simulink model "apf_offline"  (R2022b)
settings: Solver=VariableStepAuto  StartTime=0.0  StopTime=40  RelTol=1e-3
values from neighbouring files (symbols this model uses):
  d0 = 2.5    [apf_offline_script.m]
  g = 9.81    [apf_offline_script.m]
  Ib = diag([0.0347563 0.0458929 0.0977])    [apf_offline_script.m]
  initori = [0 0 0]    [scenario_generator.m]
  initpos = q_0    [scenario_generator.m]
  initvel = [0 0 0]    [scenario_generator.m]
  k_att = 0.8    [apf_offline_script.m]
  k_rep = 0.03    [apf_offline_script.m]
  kp = diag([6 6 6])    [apf_offline_script.m]
  kr = diag([2 2.3 0.15])    [apf_offline_script.m]
  kv = diag([4.7 4.7 4.7])    [apf_offline_script.m]
  kw = diag([0.4 0.52 0.18])    [apf_offline_script.m]
  mass = 1.52    [apf_offline_script.m]
  q_goal = [10 10 -10]    [apf_offline_script.m]
  q_obs1 = obs_points_gen(obs_1)    [apf_offline_script.m]
  q_obs2 = obs_points_gen(obs_2)    [apf_offline_script.m]
  q_obstacles = [obs_points_gen(obs_1); obs_points_gen(obs_2)]    [apf_offline_script.m]
  Ts = 0.001    [apf_offline_script.m]
  uT_0 = 14.92    [apf_offline_script.m]
libraries: uavsimlib x3, eeGeneralControl x1, robotcorelib x1
settings Model: VariantFading=off  Creator=The MathWorks, Inc.  LastModifiedBy=stefa
settings DebuggingCC: UnconnectedInputMsg=warning  UnconnectedOutputMsg=warning  UnconnectedLineMsg=warning
settings ModelReferenceCC: EnableRefExpFcnMdlSchedulingChecks=on
settings RTWCC: DLArmComputeVersion=19.05

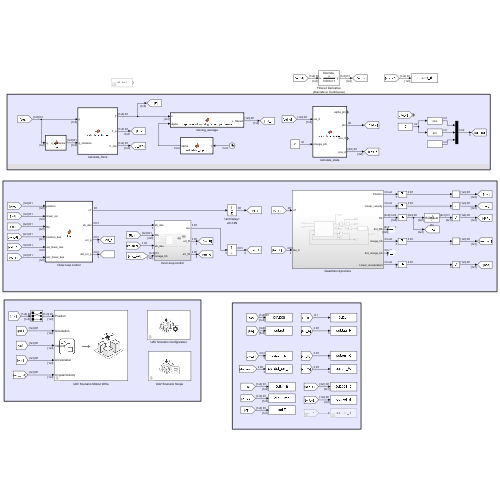
[thumbnail: Simulink's stored preview of the top-level diagram]
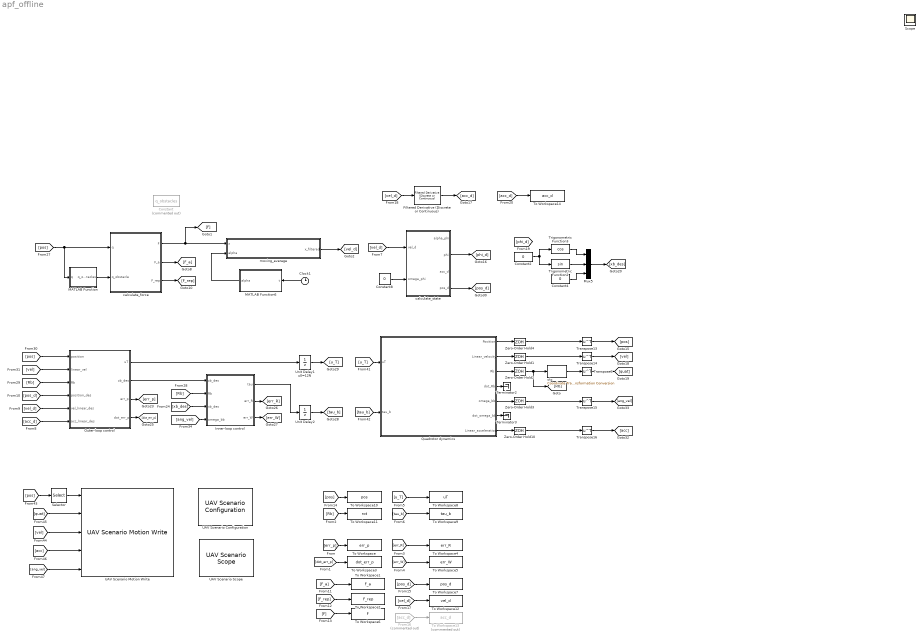
== system apf_offline ==
  Clock1 : Clock
  Constant : Constant  Commented=on  Value=q_obstacles
  Constant2 : Constant  Value=0
  Constant4 : Constant  Value=0
  Constant8 : Constant  Value=0
  Filtered Derivative (Discrete or Continuous) : eeGeneralControl/Filtered Derivative (Discrete or Continuous)  K=1  T=Ts  B=inf  A=-inf  minRatio=10  init_option=Specify as parameter  x0=[0 0 0]  Ts=-1
      settings: LibrarySourceBlock=|
      | ee_sl_lib/General Control/Filtered Derivative
      | (Discrete or Continuous)
  From16 : From  Commented=on  GotoTag=acc_d
  Inner-loop control : Subsystem
  MATLAB Function : MATLAB Function  TreatAsAtomicUnit=on
  MATLAB Function6 : MATLAB Function  TreatAsAtomicUnit=on
  Mux5 : Mux  Inputs=3
  Outer-loop control : MATLAB Function  TreatAsAtomicUnit=on
  Quadrotor dynamics : Subsystem
  Selector : Selector  InputPortWidth=3  IndexOptions=Index vector (dialog)  Indices=[2 1 3]  OutputSizes=1
  Terminator2 : Terminator
  Terminator3 : Terminator
  To Workspace : ToWorkspace  VariableName=err_p  SaveFormat=Timeseries  SampleTime=-1
  To Workspace1 : ToWorkspace  VariableName=F_a  SampleTime=-1
      settings: Save2DSignal=2-D array (concatenate along first dimension)
  To Workspace10 : ToWorkspace  VariableName=pos  SampleTime=-1
      settings: Save2DSignal=2-D array (concatenate along first dimension)
  To Workspace11 : ToWorkspace  VariableName=rot  SaveFormat=Timeseries  SampleTime=-1
  To Workspace12 : ToWorkspace  VariableName=vel_d  SampleTime=-1
      settings: Save2DSignal=2-D array (concatenate along first dimension)
  To Workspace13 : ToWorkspace  Commented=on  VariableName=acc_d  SampleTime=-1
  To Workspace14 : ToWorkspace  VariableName=acc_d  SampleTime=-1
      settings: Save2DSignal=2-D array (concatenate along first dimension)
  To Workspace2 : ToWorkspace  VariableName=F_rep  SampleTime=-1
      settings: Save2DSignal=2-D array (concatenate along first dimension)
  To Workspace3 : ToWorkspace  VariableName=dot_err_p  SaveFormat=Timeseries  SampleTime=-1
  To Workspace4 : ToWorkspace  VariableName=err_R  SaveFormat=Timeseries  SampleTime=-1
  To Workspace5 : ToWorkspace  VariableName=err_W  SaveFormat=Timeseries  SampleTime=-1
  To Workspace6 : ToWorkspace  VariableName=F  SampleTime=-1
      settings: Save2DSignal=2-D array (concatenate along first dimension)
  To Workspace7 : ToWorkspace  VariableName=pos_d  SampleTime=-1
  To Workspace8 : ToWorkspace  VariableName=uT  SaveFormat=Timeseries  SampleTime=-1
  To Workspace9 : ToWorkspace  VariableName=tau_b  SaveFormat=Timeseries  SampleTime=-1
  Transpose{6,13..16} (5 alike) : Math  Operator=transpose
  Trigonometric Function2 : Trigonometry
  Trigonometric Function3 : Trigonometry  Operator=cos
  UAV Scenario Configuration : uavsimlib/UAV Scenario Configuration  Priority=-1  UAVScenarioObject=scene  SampleTime=Ts  UpdateParam=true  SensorMotionBusName='SensorMotionBus'  PlatformMotionBusName='PlatformMotionBus'  ScenarioMotionBusName='ScenarioMotionBus'  ScenarioMotionSignalName='ScenarioMotions'
  UAV Scenario Motion Write : uavsimlib/UAV Scenario Motion Write  Priority=0  PlatName='platformUAV'  ReferenceFrame=NED
  UAV Scenario Scope : uavsimlib/UAV Scenario Scope  Priority=1  SensorNameTable={}  SampleTime=0.1
  Unit Delay1 u0=12N : UnitDelay  InitialCondition=uT_0  SampleTime=Ts
  Unit Delay2 : UnitDelay  InitialCondition=[0 0 0]  SampleTime=Ts
  Zero-Order Hold{1..4,10} (5 alike) : ZeroOrderHold  SampleTime=Ts
  calculate_force : MATLAB Function  TreatAsAtomicUnit=on
  calculate_state : MATLAB Function  TreatAsAtomicUnit=on
  ctc : robotcorelib/Coordinate Transformation Conversion  InputRepresentation=Rotation Matrix  InputEulerSequence=ZYX  ShowTrVecInputPort=on  OutputRepresentation=Quaternion  OutputEulerSequence=ZYX  ShowTrVecOutputPort=on  SimulateUsing=Interpreted execution
  moving_average : MATLAB Function  TreatAsAtomicUnit=on
  Scope : Scope
  wires:
  Trigonometric Function3/1 -> Mux5/1
  Constant4/1 -> Mux5/3
  Constant2/1 -> Trigonometric Function2/1, Trigonometric Function3/1
  Trigonometric Function2/1 -> Mux5/2
  Constant8/1 -> calculate_state/2(omega_phi)
  calculate_state/2(phi) -> [phi_d]
  MATLAB Function/1(q_obstacles) -> calculate_force/2(q_obstacle)
  calculate_force/1(F) -> [F], moving_average/1(x)
  Quadrotor dynamics/1(Position) -> Zero-Order Hold4/1
  Outer-loop control/2(zb_des) -> Inner-loop control/1(zb_des)
  Zero-Order Hold4/1 -> Transpose13/1
  Quadrotor dynamics/6(dot_omega_bb) -> Terminator3/1
  Quadrotor dynamics/5(omega_bb) -> Zero-Order Hold3/1
  [xb_des] -> Inner-loop control/3(xb_des)
  [vel_d] -> Outer-loop control/5(vel_linear_des)
  Quadrotor dynamics/4(dot_Rb) -> Terminator2/1
  Zero-Order Hold2/1 -> [Rb], ctc/1
  [acc_d] -> Outer-loop control/6(acc_linear_des)
  Inner-loop control/2(err_R) -> [err_R]
  Zero-Order Hold1/1 -> Transpose14/1
  Inner-loop control/3(err_W) -> [err_W]
  Inner-loop control/1(tau) -> Unit Delay2/1
  Unit Delay1 u0=12N/1 -> [u_T]
  Quadrotor dynamics/2(Linear_velocity) -> Zero-Order Hold1/1
  Unit Delay2/1 -> [tau_b]
  Outer-loop control/3(err_p) -> [err_p]
  Outer-loop control/1(uT) -> Unit Delay1 u0=12N/1
  [pos_d] -> Outer-loop control/4(position_des)
  Outer-loop control/4(dot_err_p) -> [dot_err_p]
  Quadrotor dynamics/3(Rb) -> Zero-Order Hold2/1
  ctc/1 -> Transpose6/1
  [pos] -> Selector/1
  [quat] -> UAV Scenario Motion Write/2
  [vel] -> UAV Scenario Motion Write/3
  Transpose6/1 -> [quat]
  [Rb] -> Inner-loop control/2(Rb)
  [Rb] -> Outer-loop control/3(Rb)
  [pos] -> Outer-loop control/1(position)
  [vel] -> Outer-loop control/2(linear_vel)
  [pos] -> MATLAB Function/1(q), calculate_force/1(q)
  calculate_state/4(pos_d) -> [pos_d]
  [vel_d] -> calculate_state/1(vel_d)
  calculate_force/3(F_rep) -> [F_rep]
  calculate_force/2(F_a) -> [F_a]
  [ang_vel] -> Inner-loop control/4(omega_bb)
  Mux5/1 -> [xb_des]
  [u_T] -> Quadrotor dynamics/1(uT)
  [tau_b] -> Quadrotor dynamics/2(tau_b)
  Transpose13/1 -> [pos]
  Transpose14/1 -> [vel]
  Transpose16/1 -> [acc]
  Zero-Order Hold10/1 -> Transpose16/1
  Quadrotor dynamics/7(Linear_acceleration) -> Zero-Order Hold10/1
  [acc] -> UAV Scenario Motion Write/4
  Zero-Order Hold3/1 -> Transpose15/1
  Transpose15/1 -> [ang_vel]
  [ang_vel] -> UAV Scenario Motion Write/5
  Clock1/1 -> MATLAB Function6/1(t)
  MATLAB Function6/1(alpha) -> moving_average/2(alpha)
  Selector/1 -> UAV Scenario Motion Write/1
  [tau_b] -> To Workspace9/1
  [err_p] -> To Workspace/1
  [pos] -> To Workspace10/1
  [dot_err_p] -> To Workspace3/1
  [u_T] -> To Workspace8/1
  [err_W] -> To Workspace5/1
  [err_R] -> To Workspace4/1
  [Rb] -> To Workspace11/1
  [F_rep] -> To Workspace2/1
  [F_a] -> To Workspace1/1
  [F] -> To Workspace6/1
  [pos_d] -> To Workspace7/1
  From16/1 -> To Workspace13/1
  [vel_d] -> To Workspace12/1
  moving_average/1(x_filtered) -> [vel_d]
  Filtered Derivative (Discrete or Continuous)/1 -> [acc_d]
  [vel_d] -> Filtered Derivative (Discrete or Continuous)/1
  [acc_d] -> To Workspace14/1

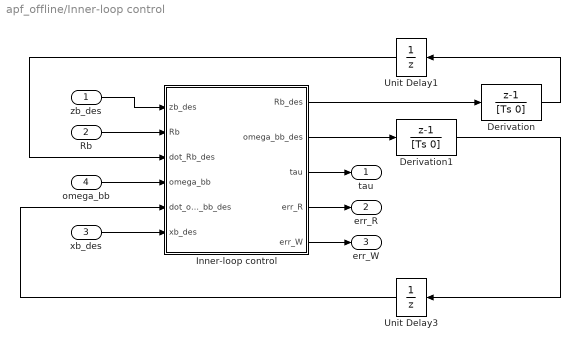
== system apf_offline/Inner-loop control ==
  zb_des : Inport
  Rb : Inport  Port=2
  xb_des : Inport  Port=3
  omega_bb : Inport  Port=4
  Derivation : DiscreteTransferFcn  Numerator=[1 -1]  Denominator=[Ts 0]  InitialStates=[1 0 0;0 1 0;0 0 1]  SampleTime=Ts
  Derivation1 : DiscreteTransferFcn  Numerator=[1 -1]  Denominator=[Ts 0]  InitialStates=[0 0 0]  SampleTime=Ts
  Inner-loop control : MATLAB Function  TreatAsAtomicUnit=on
  Unit Delay1 : UnitDelay  InitialCondition=eul2rotm(initori)  SampleTime=Ts
  Unit Delay3 : UnitDelay  InitialCondition=[0 0 0]  SampleTime=Ts
  tau : Outport
  err_R : Outport  Port=2
  err_W : Outport  Port=3
  wires:
  Derivation1/1 -> Unit Delay3/1
  Unit Delay3/1 -> Inner-loop control/5(dot_omega_bb_des)
  Inner-loop control/5(err_W) -> err_W/1
  Inner-loop control/3(tau) -> tau/1
  Derivation/1 -> Unit Delay1/1
  Inner-loop control/2(omega_bb_des) -> Derivation1/1
  Inner-loop control/1(Rb_des) -> Derivation/1
  Inner-loop control/4(err_R) -> err_R/1
  zb_des/1 -> Inner-loop control/1(zb_des)
  xb_des/1 -> Inner-loop control/6(xb_des)
  Unit Delay1/1 -> Inner-loop control/3(dot_Rb_des)
  omega_bb/1 -> Inner-loop control/4(omega_bb)
  Rb/1 -> Inner-loop control/2(Rb)

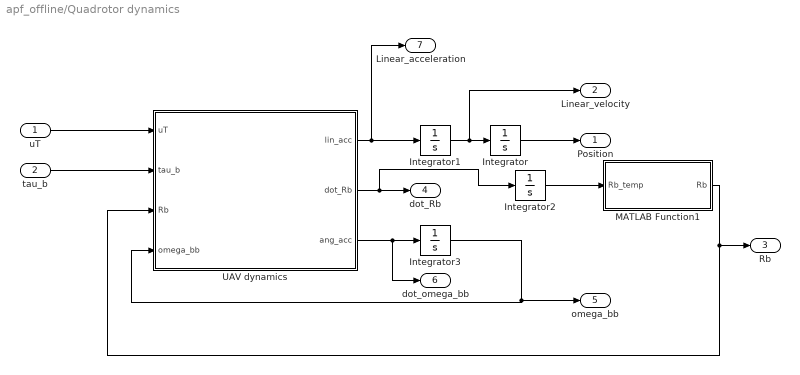
== system apf_offline/Quadrotor dynamics ==
  uT : Inport
  tau_b : Inport  Port=2
  Integrator : Integrator  InitialCondition=initpos
  Integrator1 : Integrator  InitialCondition=initvel
  Integrator2 : Integrator  InitialCondition=eul2rotm(initori)
  Integrator3 : Integrator  InitialCondition=[0 0 0]
  MATLAB Function1 : MATLAB Function  TreatAsAtomicUnit=on
  UAV dynamics : MATLAB Function  TreatAsAtomicUnit=on
  Position : Outport
  Linear_velocity : Outport  Port=2
  Rb : Outport  Port=3
  dot_Rb : Outport  Port=4
  omega_bb : Outport  Port=5
  dot_omega_bb : Outport  Port=6
  Linear_acceleration : Outport  Port=7
  wires:
  tau_b/1 -> UAV dynamics/2(tau_b)
  Integrator/1 -> Position/1
  UAV dynamics/3(ang_acc) -> dot_omega_bb/1, Integrator3/1
  UAV dynamics/1(lin_acc) -> Integrator1/1, Linear_acceleration/1
  uT/1 -> UAV dynamics/1(uT)
  Integrator1/1 -> Linear_velocity/1, Integrator/1
  Integrator3/1 -> UAV dynamics/4(omega_bb), omega_bb/1
  UAV dynamics/2(dot_Rb) -> Integrator2/1, dot_Rb/1
  MATLAB Function1/1(Rb) -> Rb/1, UAV dynamics/3(Rb)
  Integrator2/1 -> MATLAB Function1/1(Rb_temp)

== matlab function apf_offline/calculate_force ==
  data: q input; F output; q_obstacle input; q_goal parameter; F_a output; F_rep output; k_att parameter; k_rep parameter; d0 parameter
function [F, F_a, F_rep]  = calculate_force(q, q_obstacle, q_goal, k_att, k_rep, d0)

e_pos = q_goal-q;

if(norm(e_pos)<1)
    F_a = k_att * e_pos;
else
    F_a = k_att * e_pos/norm(e_pos);

end
gamma = 3;


% Inizializza la forza repulsiva
F_rep = zeros(1, 3);

%Calcola la forza repulsiva per ciascun ostacolo
for i = 1:size(q_obstacle, 1)
    q_obs = q_obstacle(i,:);
    dist = norm(q - q_obs);

    if dist <= d0
        eta_q = dist;
        eta_q0 = d0;
        grad_eta_q = (q - q_obs) / dist;

        F_rep = F_rep + (k_rep/(eta_q^2))*(1/eta_q - 1/eta_q0)^(gamma-1) * grad_eta_q;
    end
end
F = F_a + F_rep;

end

== matlab function apf_offline/MATLAB Function6 ==
  data: t input; alpha output
function alpha  = calculate_alpha(t)
    % Calcola il valore di alpha in base all'istante temporale t
    
    % Define initial and final alpha values
    alpha_initial = 0.0000005;
    alpha_final = 0.5;
    alpha_final = 0.005;
    
    % Define the time duration over which alpha should reach final value

    time_to_increase = 10;  % Increase alpha over 10 seconds
    alpha = alpha_initial * (100*t / 2)^2;

    % Calculate alpha based on a combination of slow start and faster growth
%     if t <= 2  % Slow start for the first 2 seconds
%         alpha = alpha_initial * (t / 2)^2;  % Quadratic ramp up
%     else
%         alpha = alpha_initial + (alpha_final - alpha_initial) * ((t - 2) / (time_to_increase - 2));
%     end
    
    % Ensure alpha is within bounds
    alpha = max(min(alpha, alpha_final), alpha_initial);


end

== matlab function apf_offline/calculate_state ==
  settings: updateMethod=DISCRETE
  data: alpha_phi output; vel_d input; omega_phi input; phi output; acc_d output; pos_d output; initpos parameter; initvel parameter; Ts parameter
function [alpha_phi, phi, acc_d, pos_d] = calculate_state(vel_d, omega_phi, initpos, initvel, Ts)
    % Calcola le posizioni e le accelerazioni a partire dalle velocità
    % Inizializza le variabili persistenti
    persistent x_prev y_prev z_prev phi_prev
    persistent v_x_prev v_y_prev v_z_prev omega_phi_prev

    dt = Ts;

    % Se è la prima chiamata, inizializza le variabili persistenti
    if isempty(x_prev)
        x_prev = initpos(1);
        y_prev = initpos(2);
        z_prev = initpos(3);
        phi_prev = 0;
        v_x_prev = initvel(1);
        v_y_prev = initvel(2);
        v_z_prev = initvel(3);
        omega_phi_prev = 0;
    end

    % Associo le velocità desiderate 
    v_x = vel_d(1);
    v_y = vel_d(2);
    v_z = vel_d(3);
    
    % Calcola le posizioni integrando le velocità
    x = x_prev + v_x * dt;
    y = y_prev + v_y * dt;
    z = z_prev + v_z * dt;
    phi = phi_prev + omega_phi * dt;
    
    % Calcola le accelerazioni derivando le velocità
    a_x = (v_x - v_x_prev) / dt;
    a_y = (v_y - v_y_prev) / dt;
    a_z = (v_z - v_z_prev) / dt;
    alpha_phi = (omega_phi - omega_phi_prev) / dt;
    
    % Sistema gli output
    pos_d = [x; y; z];
    acc_d = [a_x; a_y; a_z];

    % Aggiorna le variabili persistenti
    x_prev = x;
    y_prev = y;
    z_prev = z;
    phi_prev = phi;
    v_x_prev = v_x;
    v_y_prev = v_y;
    v_z_prev = v_z;
    omega_phi_prev = omega_phi;
end

== matlab function apf_offline/MATLAB Function ==
  data: q input; q_obstacles output; q_obs1 parameter; q_obs2 parameter
function q_obstacles = fcn(q, q_obs1, q_obs2)
distanza=[];
q_obstacles=[zeros(3);zeros(3)];
min=1000;
index=0;
for i=1:size(q_obs1,1)
    distanza = [distanza norm(q - q_obs1(i,:))];
    if(distanza(i) < min)
        min=distanza(i);
        index=i;
    end
end
%[M,I]= min(distanza,[],'all');
q_obs = q_obs1(index,:);

distanza2=[];
min=1000;
index=0;
for k=1:size(q_obs2,1)
    distanza2 = [distanza2 norm(q - q_obs2(k,:))];
    if(distanza2(k) < min)
        min=distanza2(k);
        index=k;
    end
end
%[M,I]= min(distanza,[],'all');
q_obstacles(1,1:3) = q_obs;
q_obstacles(2,1:3) = q_obs2(index,:);

== matlab function apf_offline/Outer-loop control ==
  data: position input size=3; uT output size=1; linear_vel input size=3; Rb input size=[3,3]; zb_des output size=3; mass parameter size=1; position_des input size=3; vel_linear_des input size=3; acc_linear_des input size=3; err_p output size=3; dot_err_p output size=3; kp parameter; kv parameter; g parameter
function [uT, zb_des, err_p, dot_err_p] = fcn(position, linear_vel, Rb, mass, ...
    position_des, vel_linear_des, acc_linear_des, kp, kv, g)

%% WRITE HERE THE OUTER-LOOP CONTROL
% position: linear position measure
% linear_vel: linear velocity measure
% Rb: current rotation matrix
% mass: mass of the UAV
% positon_des: desired linear position from the planner
% vel_linear_des: desired linear velocity from the planner
% acc_linear_des: desired linear acceleration from the planner
% ---
% uT: commanded total thrust
% zb_des: desired z-axis of the body frame
% err_p: position error
% dot_err_p: time derivative of the positon error

%% OUTER-LOOP CONTROL

err_p = position - position_des;
dot_err_p = linear_vel - vel_linear_des;


% NON SO COME CHIAMARLA se avete fantasia diamogli un nome decente
num = -kp * err_p - kv * dot_err_p - mass * g * [0; 0; 1] + mass * acc_linear_des;

uT = ((-num')* Rb * [0; 0; 1]);  

zb_des = - num / norm(num);

== matlab function apf_offline/Inner-loop control/Inner-loop control ==
  data: Rb_des output size=[3,3]; omega_bb_des output size=3; tau output size=3; zb_des input size=3; Rb input size=[3,3]; dot_Rb_des input size=[3,3]; omega_bb input size=3; dot_omega_bb_des input size=3; xb_des input size=3; Ib parameter size=[3,3]; err_R output size=3; err_W output size=3; kw parameter; kr parameter
function [Rb_des,omega_bb_des,tau,err_R,err_W] = fcn(zb_des,Rb,dot_Rb_des,omega_bb,dot_omega_bb_des,xb_des,Ib, kw, kr)

%% WRITE HERE THE INNER-LOOP CONTROL
% zb_des: desired z-axis of the body frame
% Rb: current rotation matrix
% dot_Rb_des: time-derivative of the desired rotation matrix
% omega_bb: current angular velocity expressed in the body frame
% dot_omega_bb_des: desired angular acceleration expressed in the body
% frame
% xb_des: desired x-axis of the body frame form the planner
% Ib: inertia matrix of the UAV with respect to the body frame
% ---
% Rb_des: desired rotation matrix
% omega_bb_des: desired angular velocity expressed in the body frame (given
% below as a hint)
% tau: commanded control torque
% err_R: rotational error in SO(3)
% err_W: angular velocity error in SO(3)

yb_des=( skew(zb_des) * xb_des) / norm( ( skew(zb_des) * xb_des) );

Rb_des=[skew(yb_des)*zb_des yb_des zb_des];

err_R= 1/2 * wedge( (Rb_des') * Rb - (Rb') * Rb_des);

omega_bb_des = wedge(Rb_des'*dot_Rb_des);

err_W=omega_bb - (Rb') * Rb_des * omega_bb_des; 

tau=-kr * err_R - kw * err_W + skew(omega_bb) * Ib * omega_bb - Ib * (skew(omega_bb) * (Rb') * Rb_des * omega_bb_des - (Rb') * Rb_des * dot_omega_bb_des);
end

function S = skew(v)
if(numel(v)~= 1)
S= [0 -v(3) v(2); 
    v(3) 0 -v(1);
    -v(2) v(1) 0];
else
S= zeros(3);
end
end

function v = wedge(S)
v1 = S(3,2);
v2 = S(1,3);
v3 = S(2,1);
v = [v1 v2 v3]';
end

== matlab function apf_offline/Quadrotor dynamics/MATLAB Function1 ==
  data: Rb_temp input; Rb output
function Rb = fcn(Rb_temp)
    [U,S,V] = svd(Rb_temp);
    sigma = det(U*V');
    S_ = diag([1 1 sigma]);

    Rb = U*S_*V';
end

== matlab function apf_offline/Quadrotor dynamics/UAV dynamics ==
  data: uT input size=1; tau_b input size=3; lin_acc output size=3; Rb input size=[3,3]; omega_bb input size=3; dot_Rb output size=[3,3]; ang_acc output size=3; mass parameter size=1; Ib parameter size=[3,3]
function [lin_acc, dot_Rb, ang_acc] = fcn(uT,tau_b,Rb,omega_bb,mass, Ib)

lin_acc = 9.81*[0 0 1]'-(uT/mass)*Rb*[0 0 1]';
dot_Rb = Rb*skew(omega_bb);
ang_acc = inv(Ib)*(-skew(omega_bb)*Ib*omega_bb + tau_b);

end

function S = skew(v)
if(numel(v)~= 1)
S= [0 -v(3) v(2); 
    v(3) 0 -v(1);
    -v(2) v(1) 0];
else
S= zeros(3);
end
end

== matlab function apf_offline/moving_average ==
  settings: updateMethod=DISCRETE
  data: x input; x_filtered output; alpha input
function x_filtered = exponential_moving_average_vector(x, alpha)

    % Verifica che l'input x sia un vettore colonna 3x1
    if ~isequal(size(x), [1, 3])
        error('L''input x deve essere un vettore colonna 3x1.');
    end
    
    % Inizializza la variabile persistente
    persistent x_filtered_prev
    
    % Se è la prima chiamata, inizializza la variabile persistente
    if isempty(x_filtered_prev)
        x_filtered_prev = [0 0 0];
    end
    
    % Applica il filtro a media mobile esponenziale elemento per elemento
    x_filtered = (1 - alpha) * x_filtered_prev + alpha * x;
    
    % Aggiorna la variabile persistente
    x_filtered_prev = x_filtered;
end
